simulink model "cs_rectifier_average"  (R2026a)
settings: Solver=ode15s  StopTime=460  MaxStep=0.01  RelTol=1e-6
model workspace (MAT data in the model file):
  B_base = 13
  I_base = 45000
  Ki_vdc_alpha = 0.2
  Kp_vdc_alpha = 0.005
  LGrid = [1.1 1.09999989603 1.09999958429 1.09999906509 1.09999833871 1.09999740544 1.09999626556 1.09999491937 1.09999336715 1.09999160919 1.09998964578 1.09998747721 ... (46001 elements, 1x46001)]
  LKey = [1.1 1.08 1.03 0.98 0.95 1.02 1 1.08 1.12]
  L_ts = timeseries
  L_ts.Name = 'unnamed'
  L_ts.DataInfo = tsdata.datametadata
  L_ts.DataInfo.Interpolation = tsdata.interpolation
  L_ts.DataInfo.Interpolation.Fhandle : function handle (value not decoded)
  L_ts.DataInfo.Interpolation.Name = 'linear'
  L_ts.TimeInfo = tsdata.timemetadata
  L_ts.TimeInfo.Length = 46001
  L_ts.TimeInfo.DuplicateTimes = 0
  L_ts.TimeInfo.Time_ = [0 0.01 0.02 0.03 0.04 0.05 0.06 0.07 0.08 0.09 0.1 0.11 ... (46001 elements, 46001x1)]
  L_ts.TimeInfo.Initialized = 1
  L_ts.QualityInfo = tsdata.qualmetadata
  L_ts.Data_ = [1.1 1.09999989603 1.09999958429 1.09999906509 1.09999833871 1.09999740544 1.09999626556 1.09999491937 1.09999336715 1.09999160919 1.09998964578 1.09998747721 ... (46001 elements, 1x1x46001)]
  RGrid = [0.35 0.351877050317 0.3537498692 0.35561845855 0.357482820267 0.35934295625 0.3611988684 0.363050558617 0.3648980288 0.36674128085 0.368580316667 0.37041513815 ... (46001 elements, 1x46001)]
  RKey = [0.35 0.8 0.6 0.024 0.024 0.12 0.12 0.25 0.35]
  R_ts = timeseries
  R_ts.Name = 'unnamed'
  R_ts.DataInfo = tsdata.datametadata
  R_ts.DataInfo.Interpolation = tsdata.interpolation
  R_ts.DataInfo.Interpolation.Fhandle : function handle (value not decoded)
  R_ts.DataInfo.Interpolation.Name = 'linear'
  R_ts.TimeInfo = tsdata.timemetadata
  R_ts.TimeInfo.Length = 46001
  R_ts.TimeInfo.DuplicateTimes = 0
  R_ts.TimeInfo.Time_ = [0 0.01 0.02 0.03 0.04 0.05 0.06 0.07 0.08 0.09 0.1 0.11 ... (46001 elements, 46001x1)]
  R_ts.TimeInfo.Initialized = 1
  R_ts.QualityInfo = tsdata.qualmetadata
  R_ts.Data_ = [0.35 0.351877050317 0.3537498692 0.35561845855 0.357482820267 0.35934295625 0.3611988684 0.363050558617 0.3648980288 0.36674128085 0.368580316667 0.37041513815 ... (46001 elements, 1x1x46001)]
  S_transformer = 70000000
  V_primary = 10000
  V_secondary = 1200
  Vdc_filter_a = 0.995012479193
  Vdc_filter_tau = 0.01
  Vdc_ref = 1500
  alpha0_deg = 22.1916065663
  alpha_integral_max = 57.8083934337
  alpha_integral_min = -17.1916065663
  alpha_max_deg = 80
  alpha_min_deg = 5
  avg_Ki_deg_per_Vs = 0.5
  avg_Kp_deg_per_V = 0.02
  avg_converter_tau_s = 0.05
  control_sample_time = 5e-05
  dt = 0.01
  kB = 0.000288888888889
  tGrid = [0 0.01 0.02 0.03 0.04 0.05 0.06 0.07 0.08 0.09 0.1 0.11 ... (46001 elements, 1x46001)]
  tKey = [0 5 8 12 45 70 335 420 460]
  transformer_ratio = 0.12
libraries: nesl_utility x6, fl_lib x5, ee_lib x1
(part 1 of 2)
settings Model: ModifiedByFormat=GKC3-Simulink contributors  Creator=GKC3-Simulink contributors  LastModifiedBy=GKC3-Simulink contributors
settings SimscapeCC: SimscapeNominalValues="[{\"value\":\"1\",\"unit\":\"A\"},{\"value\":\"1\",\"unit\":\"bar\"},{\"value\":\"1\",\"unit\":\"cm^2\"},{\"value\":\"1\",\"unit\":\"cm^3/s\"},{\"value\":\"1\",\"unit\":\"kJ/kg\"},{\"value\":\"1\",\"unit\":\"kW\"},{\"value\":\"1\",\"unit\":\"l\"},{\"value\":\"1\",\"unit\":\"N\"},{\"value\":\"1\",\"unit\":\"N*m\"},{\"value\":\"1\",\"unit\":\"V\"}]"  SimscapeLogType=none  SimscapeLogDataHistory=5000.0

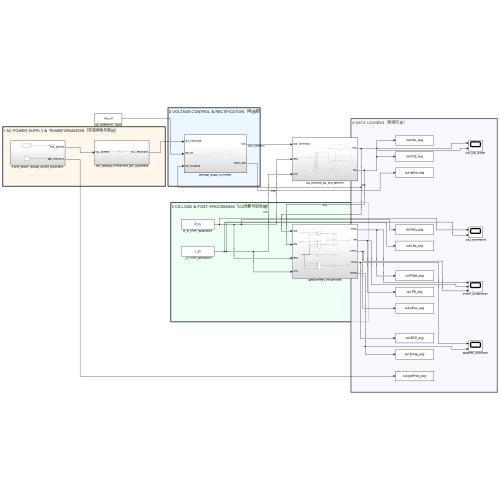
[thumbnail: Simulink's stored preview of the top-level diagram]
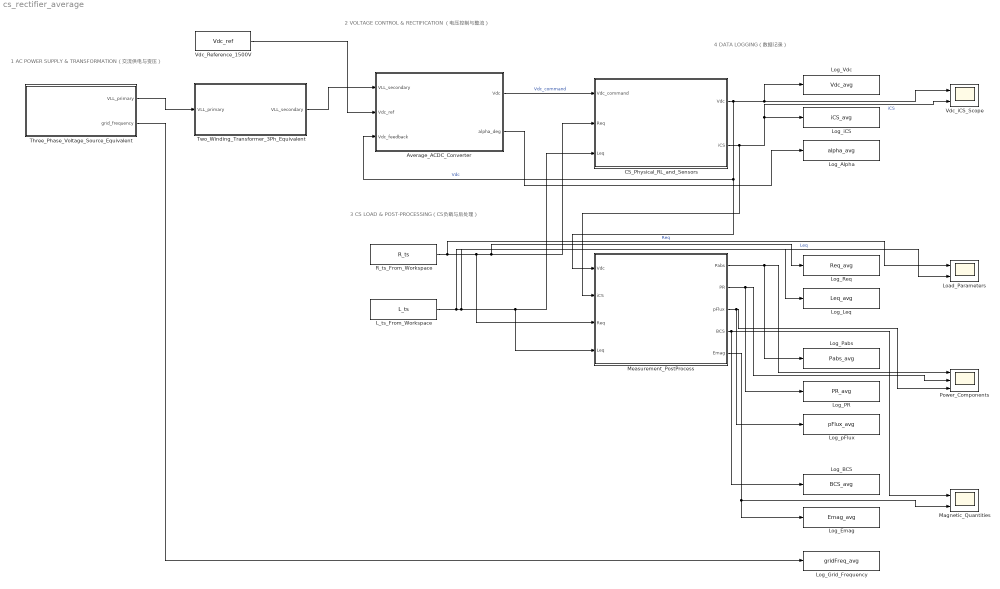
== system cs_rectifier_average ==
  note: 1 AC POWER SUPPLY & TRANSFORMATION（交流供电与变压）
  note: 2 VOLTAGE CONTROL & RECTIFICATION（电压控制与整流）
  note: 3 CS LOAD & POST-PROCESSING（CS负载与后处理）
  note: 4 DATA LOGGING（数据记录）
  Average_ACDC_Converter : Subsystem
  CS_Physical_RL_and_Sensors : Subsystem
  L_ts_From_Workspace : FromWorkspace  VariableName=L_ts
  Load_Parameters : Scope  NumInputPorts=2
  Log_Alpha : ToWorkspace  VariableName=alpha_avg  SaveFormat=Timeseries  SampleTime=-1
  Log_BCS : ToWorkspace  VariableName=BCS_avg  SaveFormat=Timeseries  SampleTime=-1
  Log_Emag : ToWorkspace  VariableName=Emag_avg  SaveFormat=Timeseries  SampleTime=-1
  Log_Grid_Frequency : ToWorkspace  VariableName=gridFreq_avg  SaveFormat=Timeseries  SampleTime=-1
  Log_Leq : ToWorkspace  VariableName=Leq_avg  SaveFormat=Timeseries  SampleTime=-1
  Log_PR : ToWorkspace  VariableName=PR_avg  SaveFormat=Timeseries  SampleTime=-1
  Log_Pabs : ToWorkspace  VariableName=Pabs_avg  SaveFormat=Timeseries  SampleTime=-1
  Log_Req : ToWorkspace  VariableName=Req_avg  SaveFormat=Timeseries  SampleTime=-1
  Log_Vdc : ToWorkspace  VariableName=Vdc_avg  SaveFormat=Timeseries  SampleTime=-1
  Log_iCS : ToWorkspace  VariableName=iCS_avg  SaveFormat=Timeseries  SampleTime=-1
  Log_pFlux : ToWorkspace  VariableName=pFlux_avg  SaveFormat=Timeseries  SampleTime=-1
  Magnetic_Quantities : Scope  NumInputPorts=2
  Measurement_PostProcess : Subsystem
  Power_Components : Scope  NumInputPorts=3
  R_ts_From_Workspace : FromWorkspace  VariableName=R_ts
  Three_Phase_Voltage_Source_Equivalent : Subsystem
  Two_Winding_Transformer_3Ph_Equivalent : Subsystem
  Vdc_Reference_1500V : Constant  Value=Vdc_ref
  Vdc_iCS_Scope : Scope  NumInputPorts=2
  wires:
  Two_Winding_Transformer_3Ph_Equivalent/1(VLL_secondary) -> Average_ACDC_Converter/1(VLL_secondary)
  Vdc_Reference_1500V/1 -> Average_ACDC_Converter/2(Vdc_ref)
  Average_ACDC_Converter/2(alpha_deg) -> Log_Alpha/1
  Three_Phase_Voltage_Source_Equivalent/1(VLL_primary) -> Two_Winding_Transformer_3Ph_Equivalent/1(VLL_primary)
  Three_Phase_Voltage_Source_Equivalent/2(grid_frequency) -> Log_Grid_Frequency/1
  Measurement_PostProcess/5(Emag) -> Magnetic_Quantities/2, Log_Emag/1
  Measurement_PostProcess/4(BCS) -> Magnetic_Quantities/1, Log_BCS/1
  Measurement_PostProcess/3(pFlux) -> Log_pFlux/1, Power_Components/3
  Measurement_PostProcess/2(PR) -> Power_Components/2, Log_PR/1
  Measurement_PostProcess/1(Pabs) -> Power_Components/1, Log_Pabs/1
  L_ts_From_Workspace/1 -> CS_Physical_RL_and_Sensors/3(Leq), Measurement_PostProcess/4(Leq), Load_Parameters/2, Log_Leq/1  "Leq"
  R_ts_From_Workspace/1 -> Log_Req/1, CS_Physical_RL_and_Sensors/2(Req), Measurement_PostProcess/3(Req), Load_Parameters/1  "Req"
  Average_ACDC_Converter/1(Vdc) -> CS_Physical_RL_and_Sensors/1(Vdc_command)  "Vdc_command"
  CS_Physical_RL_and_Sensors/1(Vdc) -> Measurement_PostProcess/1(Vdc), Average_ACDC_Converter/3(Vdc_feedback), Log_Vdc/1, Vdc_iCS_Scope/1  "Vdc"
  CS_Physical_RL_and_Sensors/2(iCS) -> Log_iCS/1, Vdc_iCS_Scope/2, Measurement_PostProcess/2(iCS)  "iCS"
